simulink model "Gr3_Ex1_3linkedRobot"  (R2024b)
settings: Solver=VariableStepAuto  StartTime=0.0  StopTime=10.0  RelTol=1e-3
values from neighbouring files (symbols this model uses):
  Kp = 100    [Gr2_Ex7_main.m]    (also in Gr2_Ex8_main.m; Gr3_Ex1_main.m = 10; Gr3_Ex2_main.m = 10)
  Kq = 10    [Gr3_Ex1_main.m]    (also in Gr3_Ex2_main.m)
  L = [1 1 0.3]    [Gr3_Ex1_main.m]    (also in Gr3_Ex2_main.m)
  qd0 = [pi/12; pi/3; pi/3]    [Gr3_Ex1_main.m]    (also in Gr3_Ex2_main.m)
  qdp = [90; -90; -90]*pi/180    [Gr3_Ex1_main.m]    (also in Gr3_Ex2_main.m)
  Xf = [1.5; -1.2]    [Gr3_Ex1_main.m]    (also in Gr3_Ex2_main.m = [1.6 0.4)
settings Model: Creator=UX434  LastModifiedBy=UX434

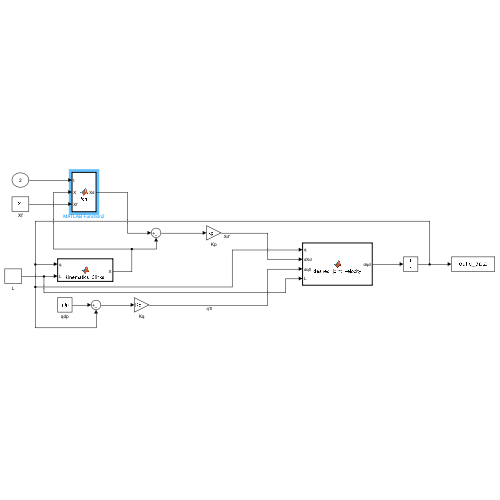
[thumbnail: Simulink's stored preview of the top-level diagram]
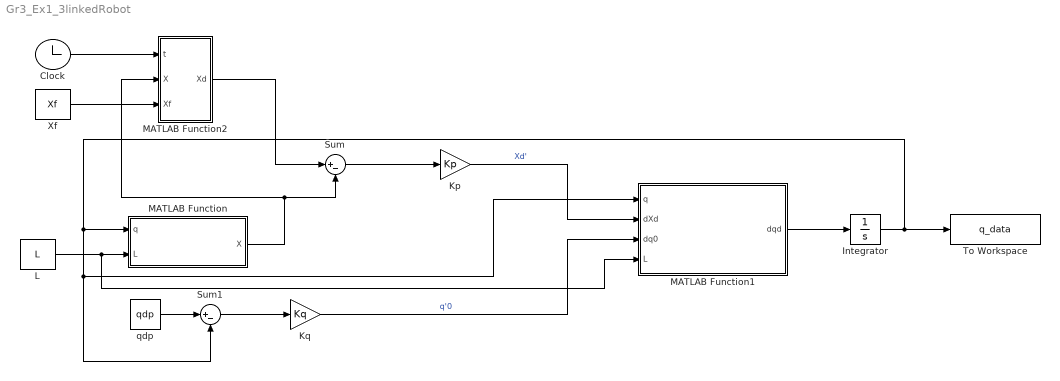
== system Gr3_Ex1_3linkedRobot ==
  Clock : Clock
  Integrator : Integrator  InitialCondition=qd0
  Kp : Gain  Gain=Kp
  Kq : Gain  Gain=Kq
  L : Constant  Value=L
  MATLAB Function : MATLAB Function  TreatAsAtomicUnit=on
  MATLAB Function1 : MATLAB Function  TreatAsAtomicUnit=on
  MATLAB Function2 : MATLAB Function  TreatAsAtomicUnit=on
  Sum : Sum  Inputs=|+-
  Sum1 : Sum  Inputs=|+-
  To Workspace : ToWorkspace  VariableName=q_data  SampleTime=-1
  Xf : Constant  Value=Xf
  qdp : Constant  Value=qdp
  wires:
  Integrator/1 -> To Workspace/1, MATLAB Function/1(q), MATLAB Function1/1(q), Sum1/2
  MATLAB Function/1(X) -> MATLAB Function2/2(X), Sum/2
  Sum/1 -> Kp/1
  Kp/1 -> MATLAB Function1/2(dXd)  "Xd'"
  qdp/1 -> Sum1/1
  Sum1/1 -> Kq/1
  Kq/1 -> MATLAB Function1/3(dq0)  "q'0"
  MATLAB Function1/1(dqd) -> Integrator/1
  Clock/1 -> MATLAB Function2/1(t)
  MATLAB Function2/1(Xd) -> Sum/1
  Xf/1 -> MATLAB Function2/3(Xf)
  L/1 -> MATLAB Function1/4(L), MATLAB Function/2(L)

== matlab function Gr3_Ex1_3linkedRobot/MATLAB Function1 ==
  data: q input; dqd output; dXd input; dq0 input; L input
function dqd = desired_joint_velocity(q, dXd, dq0, L)
    l1 = L(1);  l2 = L(2);  l3 = L(3);
    s1 = sin(q(1));  s12 = sin(q(1)+q(2));  s123 = sin(q(1)+q(2)+q(3));
    c1 = cos(q(1));  c12 = cos(q(1)+q(2));  c123 = cos(q(1)+q(2)+q(3));

    % Jacobian (2x3)
    J = [-l1*s1-l2*s12-l3*s123, -l2*s12-l3*s123, -l3*s123;
          l1*c1+l2*c12+l3*c123,  l2*c12+l3*c123,  l3*c123];

    % Pseudoinverse J# = J'*inv(J*J')
    Jp = J' / (J*J');

    % dqd = J#*dXd + (I - J#*J)*dq0
    dqd = Jp*dXd + (eye(3) - Jp*J)*dq0;
end

== matlab function Gr3_Ex1_3linkedRobot/MATLAB Function ==
  data: q input; X output; L input
function X = kinematics_3links(q, L)
    l1 = L(1);  l2 = L(2);  l3 = L(3);
    s1 = sin(q(1));  s12 = sin(q(1)+q(2));  s123 = sin(q(1)+q(2)+q(3));
    c1 = cos(q(1));  c12 = cos(q(1)+q(2));  c123 = cos(q(1)+q(2)+q(3));
    X = [l1*c1 + l2*c12 + l3*c123;
         l1*s1 + l2*s12 + l3*s123];
end

== matlab function Gr3_Ex1_3linkedRobot/MATLAB Function2 ==
  data: t input; Xd output; X input; Xf input
function Xd = fcn(t, X, Xf)
persistent X0
if isempty(X0)
    X0 = X;                     % first iteration: tip position at qi
end
s  = min(t/2, 1);               % 0 -> 1 in 2 s
Xd = [Xf(1);
      X0(2) + (Xf(2) - X0(2))*s];

% function Xd = fcn(t, X, Xf)
% persistent X0
% if isempty(X0)
%     X0 = X;                     % first iteration: tip position at qi
% end
% tp = [0, 1, 2];
% xp = [X0(1), Xf(1), Xf(1)];
% yp = [X0(2), X0(2), Xf(2)];
% s  = min(t, 2);
% Xd = [interp1(tp, xp, s); interp1(tp, yp, s)];
